simulink model "MMC_Per_arm_outer_v5_G2_tests_sat"  (R2024a)
settings: Solver=FixedStepDiscrete  StartTime=0.0  StopTime=3.2  FixedStep=Ts  RelTol=1e-3
PreLoadFcn:
  | % ---- MMC_Inner4 workspace parameters (control gains live inside the MATLAB Function blocks) ----
  | % ---------------- Converter ----------------
  | VDC     = 800;                  % DC-link voltage (V)  -> Vdc_pos / Vdc_neg = VDC/2
  | N       = 8;                    % submodules per arm
  | C       = 2.2e-3;               % submodule capacitance (F)  -> HB_xx blocks
  | vo      = 100;                  % nominal = initial capacitor voltage (V) = VDC/N  -> HB_xx, Vc_nom
  | W_nom   = 0.5*C*N*vo^2;         % nominal arm energy (J) -> initial condition of the Comm delay blocks
  | Larm    = 5e-3;                 % arm inductance (H)
  | Rarm    = 0.5;                  % arm resistance (ohm)
  | 
  | % ---------------- Grid and PCC filter ----------------
  | f       = 50;                   % grid frequency (Hz)
  | Vg_rms  = 230;                  % grid RMS voltage (V)
  | Vg_pk   = Vg_rms*sqrt(2);       % grid peak voltage (V) -> AC Voltage Source
  | Lg      = 2e-3;                 % line inductance (H)
  | Rg      = 0.1;                  % line resistance (ohm)
  | Cf      = 10e-6;                % AC filter capacitance (F)
  | Rf      = 10;                   % AC filter damping resistance (ohm)
  | 
  | % ---------------- Power set-points ----------------
  | Pstar   = 1500;                 % active-power set-point (W)
  | Qstar   = 0;                    % reactive-power set-point (var)
  | 
  | % ---------------- Timing ----------------
  | fsw     = 1250;                 % carrier frequency per submodule (Hz) -> N*fsw = 10 kHz per arm
  | Ts      = 1e-5;                 % simulation step = submodule-layer step (s)
  | Ts_ctrl = 1e-4;                 % arm-leader control step (s)
  | % ---------------- Test schedule: P* staircase and PCC load (added in _tests) ----------------
  | P_base   = 1500;                % staircase base = first level (W)
  | dP_step  = 250;                 % staircase step (W): 1500 -> 1750 -> 2000 -> 2250 -> 2500
  | t_step   = [0.6 1.0 1.4 1.8];   % step instants (s), 0.4 s hold at each level
  | t_back   = 2.2;                 % return to P_base (s) before the load test
  | P_load1  = 1000;                % PCC load 1 (W at 230 V rms)
  | P_load2  = 1000;                % PCC load 2 (W at 230 V rms)
  | R_load1  = Vg_rms^2/P_load1;    % 52.9 ohm
  | R_load2  = Vg_rms^2/P_load2;    % 52.9 ohm
  | t_load1  = 2.4;                 % Breaker load 1: closes at 2.4 s (stays closed)
  | t_load2  = [2.7 3.0];           % Breaker load 2: closes at 2.7 s, opens at 3.0 s
InitFcn:
  | % ---- MMC_Inner4 workspace parameters (control gains live inside the MATLAB Function blocks) ----
  | % ---------------- Converter ----------------
  | VDC     = 800;                  % DC-link voltage (V)  -> Vdc_pos / Vdc_neg = VDC/2
  | N       = 8;                    % submodules per arm
  | C       = 2.2e-3;               % submodule capacitance (F)  -> HB_xx blocks
  | vo      = 100;                  % nominal = initial capacitor voltage (V) = VDC/N  -> HB_xx, Vc_nom
  | W_nom   = 0.5*C*N*vo^2;         % nominal arm energy (J) -> initial condition of the Comm delay blocks
  | Larm    = 5e-3;                 % arm inductance (H)
  | Rarm    = 0.5;                  % arm resistance (ohm)
  | 
  | % ---------------- Grid and PCC filter ----------------
  | f       = 50;                   % grid frequency (Hz)
  | Vg_rms  = 230;                  % grid RMS voltage (V)
  | Vg_pk   = Vg_rms*sqrt(2);       % grid peak voltage (V) -> AC Voltage Source
  | Lg      = 2e-3;                 % line inductance (H)
  | Rg      = 0.1;                  % line resistance (ohm)
  | Cf      = 10e-6;                % AC filter capacitance (F)
  | Rf      = 10;                   % AC filter damping resistance (ohm)
  | 
  | % ---------------- Power set-points ----------------
  | Pstar   = 1500;                 % active-power set-point (W)
  | Qstar   = 0;                    % reactive-power set-point (var)
  | 
  | % ---------------- Timing ----------------
  | fsw     = 1250;                 % carrier frequency per submodule (Hz) -> N*fsw = 10 kHz per arm
  | Ts      = 1e-5;                 % simulation step = submodule-layer step (s)
  | Ts_ctrl = 1e-4;                 % arm-leader control step (s)
  | % ---------------- Test schedule: P* staircase and PCC load (added in _tests) ----------------
  | P_base   = 1500;                % staircase base = first level (W)
  | dP_step  = 250;                 % staircase step (W): 1500 -> 1750 -> 2000 -> 2250 -> 2500
  | t_step   = [0.6 1.0 1.4 1.8];   % step instants (s), 0.4 s hold at each level
  | t_back   = 2.2;                 % return to P_base (s) before the load test
  | P_load1  = 1000;                % PCC load 1 (W at 230 V rms)
  | P_load2  = 1000;                % PCC load 2 (W at 230 V rms)
  | R_load1  = Vg_rms^2/P_load1;    % 52.9 ohm
  | R_load2  = Vg_rms^2/P_load2;    % 52.9 ohm
  | t_load1  = 2.4;                 % Breaker load 1: closes at 2.4 s (stays closed)
  | t_load2  = [2.7 3.0];           % Breaker load 2: closes at 2.7 s, opens at 3.0 s
libraries: spsHalfBridgeMMCLib x16, spsSeriesRLCBranchLib x6, spsCurrentMeasurementLib x5, spsBreakerLib x2, spsGroundLib x2, spsDCVoltageSourceLib x2, spsACVoltageSourceLib x1, spspowerguiLib x1, spsVoltageMeasurementLib x1
(part 5 of 5)

== matlab function MMC_Per_arm_outer_v5_G2_tests_sat/Arm Leader UPPER/Inner Loop and Energy Balancing/B2 Energy Balancing Control ==
  data: Wo input; i_circ_ref output; Wx input; W_nom input; P_meas input; Vdc input; V_amp input; theta input; IsUpper input
function i_circ_ref = mmc_energy_balancing(Wo, Wx, W_nom, P_meas, Vdc, V_amp, theta, IsUpper)
%#codegen
% =========================================================================
% MMC_ENERGY_BALANCING  -  Block B2: total and differential arm-energy control
% -------------------------------------------------------------------------
% Block     : "B2 Energy Balancing Control" inside Inner Loop and Energy Balancing
% Rate      : Ts_ctrl = 100 us
% Instances : 2 (one per arm leader)
% Purpose   : keep the TOTAL energy of the two arms at its nominal value and
%             the DIFFERENCE between the arms at zero, by shaping the
%             circulating-current reference:
%               total energy error       -> DC component     i_dc_ref
%               differential energy error -> 50 Hz component I_dif*cos(theta)
% Inputs    : Wo       filtered own-arm energy (J)
%             Wx       filtered other-arm energy (J)
%             W_nom    nominal arm energy (J)
%             P_meas   measured active power (W), used as feed-forward
%             Vdc      DC-link voltage (V)
%             V_amp    PCC voltage amplitude (V)
%             theta    grid angle (rad)
%             IsUpper  1 for the upper arm, 0 for the lower arm
% Outputs   : i_circ_ref  circulating-current reference (A)
% =========================================================================

%% ---------------- PARAMETERS: timing ----------------
Ts = 1e-4;                               % execution period (s) = Ts_ctrl

%% ---------------- PARAMETERS: total (sum) energy loop -> DC circulating current ----------------
Kp_s     = 0.03;                         % proportional gain (A/J)
Ki_s     = 0.3;                          % integral gain (A/(J*s))
xi_s_max = 3;                            % (A) integrator limit
i_dc_max = 5;                            % (A) DC circulating-current limit

%% ---------------- PARAMETERS: differential energy loop -> 50 Hz circulating current ----------------
Kp_d      = 25;                          % proportional gain (V/J)
Ki_d      = 150;                         % integral gain (V/(J*s))
xi_d_max  = 300;                         % (V) integrator limit
I_dif_max = 3;                           % (A) amplitude limit of the 50 Hz component
V_min     = 50;                          % (V) lower bound of V_amp in the division (guard)

%% ---------------- PERSISTENT STATES ----------------
persistent xi_s xi_d                     % integrators of the sum loop (A) and of the differential loop (V)
if isempty(xi_s)                         % first call only
    xi_s = 0;                            % sum-loop integrator starts at zero
    xi_d = 0;                            % differential-loop integrator starts at zero
end

%% ---------------- 1. arm sign ----------------
if IsUpper > 0.5                         % upper arm?
    s = 1;                               % +1: the upper arm corrects in one direction...
else                                     % lower arm
    s = -1;                              % -1: ...and the lower arm in the opposite direction
end

%% ---------------- 2. total energy -> DC circulating-current component ----------------
e_sum   = 2*W_nom - (Wo + Wx);           % total energy error: nominal of both arms - (own + other) (> 0: arms need charging)
i_dc_un = P_meas/Vdc + Kp_s*e_sum + xi_s;                          % feed-forward P/Vdc (DC current the converter must draw) + PI
if abs(i_dc_un) < i_dc_max                                         % integrate only when NOT saturated (anti-windup)
    xi_s = min(max(xi_s + Ki_s*Ts*e_sum, -xi_s_max), xi_s_max);    % integrator update, clamped
end
i_dc_ref = min(max(i_dc_un, -i_dc_max), i_dc_max);                 % final clamp of the DC component

%% ---------------- 3. differential energy -> 50 Hz circulating-current component ----------------
e_dif    = Wo - Wx;                                                % energy difference own - other (J)
u_dif    = Kp_d*e_dif + xi_d;                                      % PI output as a "voltage" (V)
I_dif_un = s*u_dif/max(V_amp, V_min);                              % to a current amplitude: energy moves between arms through a 50 Hz current acting on v_ac
if abs(I_dif_un) < I_dif_max                                       % anti-windup rule
    xi_d = min(max(xi_d + Ki_d*Ts*e_dif, -xi_d_max), xi_d_max);    % integrator update, clamped
end
I_dif = min(max(I_dif_un, -I_dif_max), I_dif_max);                 % final clamp of the 50 Hz amplitude

%% ---------------- 4. circulating-current reference ----------------
i_circ_ref = i_dc_ref + I_dif*cos(theta);                          % DC component + 50 Hz component in phase with v_ac
end

== matlab function MMC_Per_arm_outer_v5_G2_tests_sat/Arm Leader UPPER/Inner Loop and Energy Balancing/B3 Inner Current Control ==
  data: i_ac_ref input; i_ref output; i_circ_ref input; i_arm input; IsUpper input; v_pi output
function [i_ref, v_pi] = mmc_inner_current(i_ac_ref, i_circ_ref, i_arm, IsUpper)
%#codegen
% =========================================================================
% MMC_INNER_CURRENT  -  Block B3: arm-current controller (PI + resonant)
% -------------------------------------------------------------------------
% Block     : "B3 Inner Current Control" inside Inner Loop and Energy Balancing
% Rate      : Ts_ctrl = 100 us
% Instances : 2 (one per arm leader)
% Purpose   : build the arm-current reference (half of the grid current +
%             the circulating current) and track it with:
%               PI            -> DC and slow components
%               resonant 50 Hz -> zero error at the grid frequency
%               resonant 100 Hz (CCSC) -> suppresses the natural 2nd-harmonic
%                                         circulating current of the MMC
% Inputs    : i_ac_ref    grid-current reference (A)
%             i_circ_ref  circulating-current reference (A)
%             i_arm       measured arm current (A)
%             IsUpper     1 for the upper arm, 0 for the lower arm
% Outputs   : i_ref       arm-current reference (A), for monitoring
%             v_pi        controller output voltage (V)
% =========================================================================

%% ---------------- PARAMETERS: timing and grid ----------------
Ts = 1e-4;                               % execution period (s) = Ts_ctrl
w0 = 2*pi*50;                            % grid angular frequency (rad/s)

%% ---------------- PARAMETERS: PI + resonant 50 Hz ----------------
Kp_i     = 12;                           % proportional gain (V/A)
Ki_i     = 1200;                         % integral gain (V/(A*s))
Kr_i     = 300;                          % resonant gain at 50 Hz (V/(A*s))
xi_i_max = 300;                          % (V) integrator limit
xr_max   = 200;                          % (V) limit of the 50 Hz resonant state
v_pi_max = 400;                          % (V) controller output limit

%% ---------------- PARAMETERS: CCSC resonant 100 Hz ----------------
USE_CCSC = true;                         % true: enable the 2nd-harmonic circulating-current suppressor
Kr_2     = 300;                          % resonant gain at 100 Hz (V/(A*s))
xr2_max  = 150;                          % (V) limit of the 100 Hz resonant state

%% ---------------- PERSISTENT STATES ----------------
persistent xi_i xr1 xr2 xc1 xc2          % integrator, 50 Hz resonator (2 states), 100 Hz resonator (2 states)
if isempty(xi_i)                         % first call only
    xi_i = 0;                            % integrator (V)
    xr1  = 0;                            % 50 Hz resonator, output state (V)
    xr2  = 0;                            % 50 Hz resonator, internal state (V)
    xc1  = 0;                            % 100 Hz resonator, output state (V)
    xc2  = 0;                            % 100 Hz resonator, internal state (V)
end

%% ---------------- 1. arm sign ----------------
if IsUpper > 0.5                         % upper arm?
    s = 1;                               % upper arm carries +i_ac/2
else                                     % lower arm
    s = -1;                              % lower arm carries -i_ac/2
end

%% ---------------- 2. arm-current reference and error ----------------
i_ref = s*0.5*i_ac_ref + i_circ_ref;     % each arm carries half the grid current (opposite signs) + the same circulating current
err_i = i_ref - i_arm;                   % current error (A)

%% ---------------- 3. integral term ----------------
xi_i = min(max(xi_i + Ki_i*Ts*err_i, -xi_i_max), xi_i_max);        % integrator update, clamped

%% ---------------- 4. resonant term at 50 Hz (symplectic Euler) ----------------
xr1 = xr1 + Ts*(Kr_i*err_i - w0*xr2);    % oscillator driven by the error -> very high gain at exactly 50 Hz
xr2 = xr2 + Ts*w0*xr1;                   % second oscillator state
xr1 = min(max(xr1, -xr_max), xr_max);    % safety clamp of the resonant output

%% ---------------- 5. resonant term at 100 Hz (CCSC) ----------------
if USE_CCSC                              % suppressor enabled?
    xc1 = xc1 + Ts*(Kr_2*err_i - 2*w0*xc2);                        % oscillator at 2*w0 driven by the error
    xc2 = xc2 + Ts*2*w0*xc1;                                       % second oscillator state
    xc1 = min(max(xc1, -xr2_max), xr2_max);                        % safety clamp
end                                      % when disabled the states simply stay at zero

%% ---------------- 6. controller output ----------------
v_pi = min(max(Kp_i*err_i + xi_i + xr1 + xc1, -v_pi_max), v_pi_max);   % P + I + R50 + R100, clamped to +/- v_pi_max
end

== matlab function MMC_Per_arm_outer_v5_G2_tests_sat/Arm Leader UPPER/Inner Loop and Energy Balancing/B4 Arm Voltage Modulation ==
  data: v_ac input; m_arm output; v_pi input; IsUpper input; Vdc input; Vc_arm input; Vc_nom input; i_ref input; i_circ_ref input; Wo input; Wx input; dbg output
function [m_arm, dbg] = mmc_arm_modulation(v_ac, v_pi, IsUpper, Vdc, Vc_arm, Vc_nom, i_ref, i_circ_ref, Wo, Wx)
%#codegen
% =========================================================================
% MMC_ARM_MODULATION  -  Block B4: arm voltage reference -> modulation index
% -------------------------------------------------------------------------
% Block     : "B4 Arm Voltage Modulation" inside Inner Loop and Energy Balancing
% Rate      : Ts_ctrl = 100 us
% Instances : 2 (one per arm leader)
% Purpose   : convert the required arm voltage into the modulation index
%             m_arm in [0, 1] that is broadcast to the submodules.
%               upper arm: v_arm = Vdc/2 - v_ac - v_pi
%               lower arm: v_arm = Vdc/2 + v_ac - v_pi
% Inputs    : v_ac     PCC voltage (V)
%             v_pi     current-controller output (V)
%             IsUpper  1 for the upper arm, 0 for the lower arm
%             Vdc      DC-link voltage (V)
%             Vc_arm   N x 1 capacitor voltages of the arm (V)
%             Vc_nom   nominal capacitor voltage (V)
%             i_ref, i_circ_ref, Wo, Wx   pass-through signals, DEBUG ONLY
% Outputs   : m_arm    arm modulation index in [0, 1]
%             dbg      5 x 1 debug vector = [i_ref; i_circ_ref; v_arm_ref; Wo; Wx]
% =========================================================================

%% ---------------- PARAMETERS ----------------
N          = 8;                          % submodules per arm
stack_min  = 0.5;                        % lower bound of the available stack voltage, as a fraction of N*Vc_nom (division guard)

%% ---------------- 1. arm sign ----------------
if IsUpper > 0.5                         % upper arm?
    s = 1;                               % upper arm: subtract v_ac
else                                     % lower arm
    s = -1;                              % lower arm: add v_ac
end

%% ---------------- 2. required arm voltage ----------------
v_arm_ref = Vdc/2 - s*v_ac - v_pi;       % half the DC link, minus the grid voltage (with arm sign), minus the controller correction

%% ---------------- 3. available stack voltage ----------------
V_stack = max(sum(Vc_arm), stack_min*N*Vc_nom);                    % sum of the N capacitor voltages, floored to avoid dividing by a small number

%% ---------------- 4. modulation index ----------------
m_arm = min(max(v_arm_ref/V_stack, 0), 1);                         % required / available, clamped to [0, 1] -> sent to the submodules

%% ---------------- 5. debug vector (monitoring only) ----------------
dbg = [i_ref; i_circ_ref; v_arm_ref; Wo; Wx];                      % unpacked at the root level by "Demux dbg UP"
end

== matlab function MMC_Per_arm_outer_v5_G2_tests_sat/SM_u2/Neighbors ==
  data: Vc_arm input; Vc_i output; i input; Vc_prev output; Vc_next output
function [Vc_i, Vc_prev, Vc_next] = get_neighbors(Vc_arm, i)
%#codegen
% =========================================================================
% GET_NEIGHBORS  -  Ring-link emulation for submodule number i
% -------------------------------------------------------------------------
% Block     : "Neighbors" inside every SM_ux / SM_lx subsystem
% Rate      : Ts = 10 us
% Instances : 16 (one per submodule)
% Purpose   : in simulation the whole capacitor-voltage vector of the arm is
%             available, but a real submodule only knows its OWN voltage and
%             the voltages of its two ring neighbours. This block hides
%             everything else, so the local controller stays truly local.
% Inputs    : Vc_arm  N x 1 vector of capacitor voltages of the arm (V)
%             i       own submodule index, 1..N
% Outputs   : Vc_i    own capacitor voltage (V)
%             Vc_prev voltage of the previous ring neighbour (V)
%             Vc_next voltage of the next ring neighbour (V)
% =========================================================================

%% ---------------- PARAMETERS ----------------
N = 8;                                   % submodules per arm (= length of Vc_arm, the Mux of the 8 HB voltages)

%% ---------------- 1. own index, made safe ----------------
k = min(max(round(i), 1), N);            % round to an integer and clamp to [1, N] (protects against a bad sm_id)

%% ---------------- 2. own voltage ----------------
Vc_i = Vc_arm(k);                        % own capacitor voltage

%% ---------------- 3. ring neighbours (circular: SM1 and SMN are neighbours) ----------------
if k == 1                                % first submodule of the ring
    Vc_prev = Vc_arm(N);                 % previous neighbour wraps around to the last submodule
    Vc_next = Vc_arm(2);                 % next neighbour is SM2
elseif k == N                            % last submodule of the ring
    Vc_prev = Vc_arm(N - 1);             % previous neighbour is SM(N-1)
    Vc_next = Vc_arm(1);                 % next neighbour wraps around to SM1
else                                     % any submodule in the middle
    Vc_prev = Vc_arm(k - 1);             % previous neighbour
    Vc_next = Vc_arm(k + 1);             % next neighbour
end
end

== matlab function MMC_Per_arm_outer_v5_G2_tests_sat/SM_u2/Local Ctrl ==
  data: sm_id input; S_top output; m_arm input; i_arm input; Vc_i input; Vc_prev input; Vc_next input; t input; S_bot output
function [S_top, S_bot] = hb_sm_local_ctrl(sm_id, m_arm, i_arm, Vc_i, Vc_prev, Vc_next, t)
%#codegen
% =========================================================================
% HB_SM_LOCAL_CTRL  -  Submodule local controller: neighbour balancing + PSC-PWM
% -------------------------------------------------------------------------
% Block     : "Local Ctrl" inside every SM_ux / SM_lx subsystem
% Rate      : Ts = 10 us
% Instances : 16 (one per half-bridge submodule)
% Purpose   : decide the two gate signals of ONE half-bridge submodule using
%             only local information: own capacitor voltage, the two ring
%             neighbours, the arm modulation index sent by the arm leader,
%             the arm-current direction and the time base.
%             No sorting and no access to the full capacitor-voltage vector.
% Inputs    : sm_id    own index 1..N (sets the carrier phase shift)
%             m_arm    arm modulation index from the arm leader, in [0, 1]
%             i_arm    arm current (A), only its direction is used
%             Vc_i     own capacitor voltage (V)
%             Vc_prev  previous ring neighbour voltage (V)
%             Vc_next  next ring neighbour voltage (V)
%             t        simulation time (s), carrier time base
% Outputs   : S_top    upper switch gate (1 = on)  -> capacitor INSERTED (+Vc)
%             S_bot    lower switch gate (1 = on)  -> capacitor BYPASSED (0 V)
% =========================================================================

%% ---------------- PARAMETERS ----------------
N      = 8;                              % submodules per arm -> carrier phase shift of SM k = (k-1)/N of a period
fsw    = 1250;                           % carrier frequency per submodule (Hz) -> N*fsw = 10 kHz apparent arm ripple
k_v    = 0.2;                            % balancing gain (1/V): modulation-index change per volt of error
dead   = 0.1;                            % dead-band (V): errors smaller than this are ignored (no chattering)
Iscale = 1.0;                            % current scale (A) of the smooth sign function tanh(i_arm/Iscale)

%% ---------------- 1. neighbour-average balancing correction ----------------
err  = 0.5*(Vc_prev + Vc_next) - Vc_i;   % error = neighbour average - own voltage (> 0: I am too low, I need charging)
if abs(err) < dead                       % error inside the dead-band?
    err = 0;                             % ignore it
end
dirn = tanh(i_arm / Iscale);             % smooth current direction in (-1, +1); > 0 means inserting CHARGES the capacitor
dm   = k_v * err * dirn;                 % correction: insert more if charging is needed AND the current charges, less otherwise
m_i  = min(max(m_arm + dm, 0), 1);       % own modulation index = arm index + correction, clamped to [0, 1]

%% ---------------- 2. phase-shifted triangular carrier (0 -> 1 -> 0) ----------------
tau = mod(t*fsw + (sm_id - 1)/N, 1);     % position inside the carrier period, in [0, 1), shifted by (sm_id-1)/N
car = 1 - abs(2*tau - 1);                % triangle: rises 0 -> 1 on the first half, falls 1 -> 0 on the second half

%% ---------------- 3. half-bridge gating ----------------
if m_i >= car                            % modulation index above the carrier?
    S_top = 1;                           % upper switch on  -> capacitor inserted (+Vc on the arm)
    S_bot = 0;                           % lower switch off
else                                     % modulation index below the carrier
    S_top = 0;                           % upper switch off
    S_bot = 1;                           % lower switch on  -> capacitor bypassed (0 V)
end
end

== matlab function MMC_Per_arm_outer_v5_G2_tests_sat/SM_l2/Neighbors ==
  data: Vc_arm input; Vc_i output; i input; Vc_prev output; Vc_next output
function [Vc_i, Vc_prev, Vc_next] = get_neighbors(Vc_arm, i)
%#codegen
% =========================================================================
% GET_NEIGHBORS  -  Ring-link emulation for submodule number i
% -------------------------------------------------------------------------
% Block     : "Neighbors" inside every SM_ux / SM_lx subsystem
% Rate      : Ts = 10 us
% Instances : 16 (one per submodule)
% Purpose   : in simulation the whole capacitor-voltage vector of the arm is
%             available, but a real submodule only knows its OWN voltage and
%             the voltages of its two ring neighbours. This block hides
%             everything else, so the local controller stays truly local.
% Inputs    : Vc_arm  N x 1 vector of capacitor voltages of the arm (V)
%             i       own submodule index, 1..N
% Outputs   : Vc_i    own capacitor voltage (V)
%             Vc_prev voltage of the previous ring neighbour (V)
%             Vc_next voltage of the next ring neighbour (V)
% =========================================================================

%% ---------------- PARAMETERS ----------------
N = 8;                                   % submodules per arm (= length of Vc_arm, the Mux of the 8 HB voltages)

%% ---------------- 1. own index, made safe ----------------
k = min(max(round(i), 1), N);            % round to an integer and clamp to [1, N] (protects against a bad sm_id)

%% ---------------- 2. own voltage ----------------
Vc_i = Vc_arm(k);                        % own capacitor voltage

%% ---------------- 3. ring neighbours (circular: SM1 and SMN are neighbours) ----------------
if k == 1                                % first submodule of the ring
    Vc_prev = Vc_arm(N);                 % previous neighbour wraps around to the last submodule
    Vc_next = Vc_arm(2);                 % next neighbour is SM2
elseif k == N                            % last submodule of the ring
    Vc_prev = Vc_arm(N - 1);             % previous neighbour is SM(N-1)
    Vc_next = Vc_arm(1);                 % next neighbour wraps around to SM1
else                                     % any submodule in the middle
    Vc_prev = Vc_arm(k - 1);             % previous neighbour
    Vc_next = Vc_arm(k + 1);             % next neighbour
end
end

== matlab function MMC_Per_arm_outer_v5_G2_tests_sat/SM_l2/Local Ctrl ==
  data: sm_id input; S_top output; m_arm input; i_arm input; Vc_i input; Vc_prev input; Vc_next input; t input; S_bot output
function [S_top, S_bot] = hb_sm_local_ctrl(sm_id, m_arm, i_arm, Vc_i, Vc_prev, Vc_next, t)
%#codegen
% =========================================================================
% HB_SM_LOCAL_CTRL  -  Submodule local controller: neighbour balancing + PSC-PWM
% -------------------------------------------------------------------------
% Block     : "Local Ctrl" inside every SM_ux / SM_lx subsystem
% Rate      : Ts = 10 us
% Instances : 16 (one per half-bridge submodule)
% Purpose   : decide the two gate signals of ONE half-bridge submodule using
%             only local information: own capacitor voltage, the two ring
%             neighbours, the arm modulation index sent by the arm leader,
%             the arm-current direction and the time base.
%             No sorting and no access to the full capacitor-voltage vector.
% Inputs    : sm_id    own index 1..N (sets the carrier phase shift)
%             m_arm    arm modulation index from the arm leader, in [0, 1]
%             i_arm    arm current (A), only its direction is used
%             Vc_i     own capacitor voltage (V)
%             Vc_prev  previous ring neighbour voltage (V)
%             Vc_next  next ring neighbour voltage (V)
%             t        simulation time (s), carrier time base
% Outputs   : S_top    upper switch gate (1 = on)  -> capacitor INSERTED (+Vc)
%             S_bot    lower switch gate (1 = on)  -> capacitor BYPASSED (0 V)
% =========================================================================

%% ---------------- PARAMETERS ----------------
N      = 8;                              % submodules per arm -> carrier phase shift of SM k = (k-1)/N of a period
fsw    = 1250;                           % carrier frequency per submodule (Hz) -> N*fsw = 10 kHz apparent arm ripple
k_v    = 0.2;                            % balancing gain (1/V): modulation-index change per volt of error
dead   = 0.1;                            % dead-band (V): errors smaller than this are ignored (no chattering)
Iscale = 1.0;                            % current scale (A) of the smooth sign function tanh(i_arm/Iscale)

%% ---------------- 1. neighbour-average balancing correction ----------------
err  = 0.5*(Vc_prev + Vc_next) - Vc_i;   % error = neighbour average - own voltage (> 0: I am too low, I need charging)
if abs(err) < dead                       % error inside the dead-band?
    err = 0;                             % ignore it
end
dirn = tanh(i_arm / Iscale);             % smooth current direction in (-1, +1); > 0 means inserting CHARGES the capacitor
dm   = k_v * err * dirn;                 % correction: insert more if charging is needed AND the current charges, less otherwise
m_i  = min(max(m_arm + dm, 0), 1);       % own modulation index = arm index + correction, clamped to [0, 1]

%% ---------------- 2. phase-shifted triangular carrier (0 -> 1 -> 0) ----------------
tau = mod(t*fsw + (sm_id - 1)/N, 1);     % position inside the carrier period, in [0, 1), shifted by (sm_id-1)/N
car = 1 - abs(2*tau - 1);                % triangle: rises 0 -> 1 on the first half, falls 1 -> 0 on the second half

%% ---------------- 3. half-bridge gating ----------------
if m_i >= car                            % modulation index above the carrier?
    S_top = 1;                           % upper switch on  -> capacitor inserted (+Vc on the arm)
    S_bot = 0;                           % lower switch off
else                                     % modulation index below the carrier
    S_top = 0;                           % upper switch off
    S_bot = 1;                           % lower switch on  -> capacitor bypassed (0 V)
end
end
